simulink model "SMC"  (R2023a)
settings: Solver=VariableStepAuto  StartTime=0.0  StopTime=10.0  RelTol=1e-3
values from neighbouring files (symbols this model uses):
  SMC_lambda = 0    [load_smc.m]
  SMC_Phi = 1.0    (= 1)    [load_smc.m]
  SMC_Tf = 0.005    [load_smc.m]
  Ts_ctrl = J.Ts_ctrl    [load_smc.m]
undefined symbols (not defined in the file or in its folder): DiscIntNeverNeededParam, Tdref_ay_bp_ms2, Tdref_table, Tdref_v_bp_ms
settings Model: Creator=Tan_Tram  LastModifiedBy=Tan_Tram

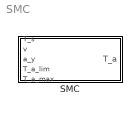
== system SMC ==
  SMC : Subsystem

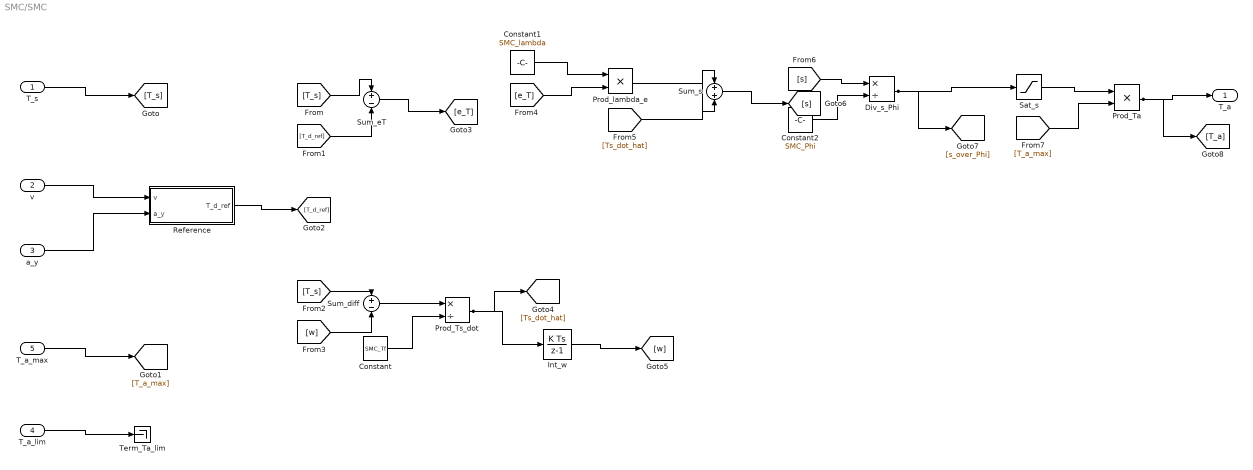
== system SMC/SMC ==
  T_s : Inport
  v : Inport  Port=2
  a_y : Inport  Port=3
  T_a_lim : Inport  Port=4
  T_a_max : Inport  Port=5
  Constant : Constant  Value=SMC_Tf
  Constant1 : Constant  Value=SMC_lambda
  Constant2 : Constant  Value=SMC_Phi
  Div_s_Phi : Product  Inputs=*/
  Int_w : DiscreteIntegrator  gainval=1  SampleTime=Ts_ctrl  ICPrevOutput=DiscIntNeverNeededParam  ICPrevScaledInput=DiscIntNeverNeededParam
  Prod_Ta : Product  Inputs=**
  Prod_Ts_dot : Product  Inputs=*/
  Prod_lambda_e : Product  Inputs=**
  Reference : Subsystem
  Sat_s : Saturate  UpperLimit=1  LowerLimit=-1
  Sum_diff : Sum  Inputs=+-
  Sum_eT : Sum  Inputs=+-
  Sum_s : Sum
  Term_Ta_lim : Terminator
  T_a : Outport
  wires:
  T_s/1 -> [T_s]
  T_a_max/1 -> [T_a_max]
  T_a_lim/1 -> Term_Ta_lim/1
  v/1 -> Reference/1(v)
  a_y/1 -> Reference/2(a_y)
  Reference/1(T_d_ref) -> [T_d_ref]
  [T_s] -> Sum_eT/1
  [T_d_ref] -> Sum_eT/2
  Sum_eT/1 -> [e_T]
  [T_s] -> Sum_diff/1
  [w] -> Sum_diff/2
  Sum_diff/1 -> Prod_Ts_dot/1
  Constant/1 -> Prod_Ts_dot/2
  Prod_Ts_dot/1 -> [Ts_dot_hat], Int_w/1
  Int_w/1 -> [w]
  Constant1/1 -> Prod_lambda_e/1
  [e_T] -> Prod_lambda_e/2
  [Ts_dot_hat] -> Sum_s/1
  Prod_lambda_e/1 -> Sum_s/2
  Sum_s/1 -> [s]
  [s] -> Div_s_Phi/1
  Constant2/1 -> Div_s_Phi/2
  Div_s_Phi/1 -> [s_over_Phi], Sat_s/1
  Sat_s/1 -> Prod_Ta/1
  [T_a_max] -> Prod_Ta/2
  Prod_Ta/1 -> T_a/1, [T_a]

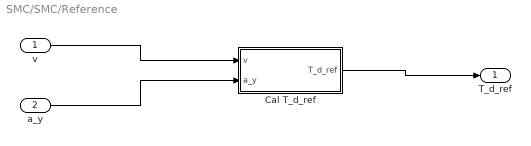
== system SMC/SMC/Reference ==
  v : Inport
  a_y : Inport  Port=2
  Cal T_d_ref : Subsystem
  T_d_ref : Outport
  wires:
  Cal T_d_ref/1(T_d_ref) -> T_d_ref/1
  a_y/1 -> Cal T_d_ref/2(a_y)
  v/1 -> Cal T_d_ref/1(v)

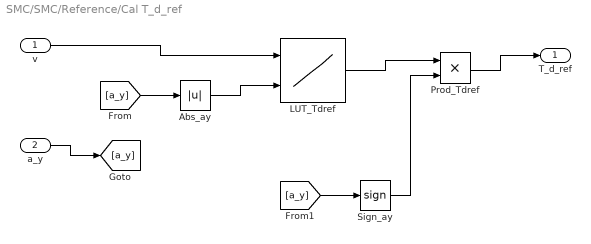
== system SMC/SMC/Reference/Cal T_d_ref ==
  v : Inport
  a_y : Inport  Port=2
  Abs_ay : Abs  SaturateOnIntegerOverflow=off
  LUT_Tdref : Lookup_n-D  BreakpointsForDimension1=Tdref_v_bp_ms  BreakpointsForDimension2=Tdref_ay_bp_ms2  Table=Tdref_table  ExtrapMethod=Clip  InternalRulePriority=Speed  RndMeth=Simplest
      settings: InputPortMap=u0,u1
  Prod_Tdref : Product  Inputs=**
  Sign_ay : Signum
  T_d_ref : Outport
  wires:
  Prod_Tdref/1 -> T_d_ref/1
  Sign_ay/1 -> Prod_Tdref/2
  LUT_Tdref/1 -> Prod_Tdref/1
  [a_y] -> Sign_ay/1
  Abs_ay/1 -> LUT_Tdref/2
  [a_y] -> Abs_ay/1
  v/1 -> LUT_Tdref/1
  a_y/1 -> [a_y]
